simulink model "FOC"  (R2024b)
settings: Solver=FixedStepDiscrete  StartTime=0.0  StopTime=0.1  FixedStep=0.00005  RelTol=1e-3  EnableMultiTasking=on
InitFcn:
  | % Check we are building from the correct Build folder
  | expectedDir = 'FOC\Build';
  | currentDir  = pwd;
  | 
  | if ~contains(currentDir, expectedDir)
  |     error(['Wrong folder! You must run from the Build folder.' ...
  |            '\nCurrent: %s' ...
  |            '\nExpected path to contain: %s'], ...
  |            currentDir, expectedDir);
  | end
  | 
  | % Load all signals and parameters
  | loadall();
values from neighbouring files (symbols this model uses):
  RNTCBreakpoints = single([      534 546 559 572 585 599 613 628 643 658 674 690      707 724 742 760 779 798 818 838 860 881 904 927      951 975 1001 1027 1054 1081 1110 1139 1170 1201 1234 1267      1302 1337 1374 1412 1451 1492 1534 1577 1622 1668 1716 1765      1817 1869 1924 1981 2039 2100 2163 2227 2295 2364 2436 2511      2588 2668 2751 2837 2927 3019 3115 3215 3318 3425 3536 3651      3771 3895 4024 4158 42 ...(+565 chars)    [maps.m]
  TNTCTable = single([      125 124 123 122 121 120 119 118 117 116 115 114      113 112 111 110 109 108 107 106 105 104 103 102      101 100 99 98 97 96 95 94 93 92 91 90      89 88 87 86 85 84 83 82 81 80 79 78      77 76 75 74 73 72 71 70 69 68 67 66      65 64 63 62 61 60 59 58 57 56 55 54      53 52 51 50 49 48 47 46 45 44 43 42      41 40 39 38 37 36 35 34 33 32 31 30      29 28 27 26 25 24 23 22 21 20 19 ...(+227 chars)    [maps.m]
undefined symbols (not defined in the file or in its folder): BEnableLedBlink, BEnableMotor, BUseEstimatedPhaseW, fClockFrequency, fElectrical, ISoftwareOCPTrip, NADCCurrentGain, NADCOffsetPhaseU, NADCOffsetPhaseV, NADCOffsetPhaseW, VOpenLoopVoltage
libraries: simulink x8, stm32f4xxblockslib x5, stm32g4xxblockslib x2, stm32blockslib x1, myLib x1, simulink_extras x1
settings Model: STM32="{\"AnalogInput\":[{\"ID\":\"FOC:8\"},{\"ID\":\"FOC:615\"},{\"ID\":\"FOC:616\"}],\"TimerBlock\":{\"ID\":\"FOC:63\"},\"HardwareInterrupt\":{\"ID\":\"FOC:599\"},\"DigitalPortRead\":{\"ID\":\"FOC:54\"},\"DigitalPortWrite\":{\"ID\":\"FOC:6\"},\"PWMOutput\":{\"ID\":\"FOC:422\"}}"  Creator=sakee  LastModifiedBy=sakee
settings SolverCC: PositivePriorityOrder=on  AutoInsertRateTranBlk=on
settings OptimizationCC: EnhancedBackFolding=on  PassReuseOutputArgsAs=Individual arguments  ZeroExternalMemoryAtStartup=off  ZeroInternalMemoryAtStartup=off  MaxStackSize=512  OptimizeBlockOrder=speed  DifferentSizesBufferReuse=on  OptimizationCustomize=off  EfficientTunableParamExpr=on
settings DebuggingCC: MultiTaskDSMMsg=none  ParameterTunabilityLossMsg=error
settings HardwareCC: ProdBitPerPointer=32  ProdBitPerSizeT=32  ProdBitPerPtrDiffT=32  ProdLargestAtomicInteger=Long  ProdLargestAtomicFloat=Double  ProdWordSize=32  ProdLongLongMode=on  ProdHWDeviceType=ARM Compatible->ARM Cortex-M
settings SFSimCC: SimCustomInitializer=CurrentSense_EnableOPAMPs();  MATLABDynamicMemAlloc=off
settings SFSimCC: SimCustomHeaderCode=|
  | #include "task_profiler.h"
  | #include "current_sense_init.h"
settings SFSimCC: SimUserSources=|
  | task_profiler.c
  | current_sense_init.c
settings SFSimCC: SimUserIncludeDirs=|
  | Execution_time
  | Current_sensing
settings RTWCC: Description=Embedded Coder  SystemTargetFile=ert.tlc  HardwareBoard=STM32G4xx Based  TLCOptions="-aInlineSetEventsForThisBaseRateFcn=TLC_FALSE -aSuppressMultiTaskScheduler=TLC_FALSE   -aRateBasedStepFcn=1"  TemplateMakefile=ert_default_tmf  RTWUseSimCustomCode=on  CustomInitializer=CurrentSense_EnableOPAMPs();  Toolchain=GNU Tools for ARM Embedded Processors  BuildConfiguration=Debug
settings RTWCC: CustomHeaderCode=|
  | #include "task_profiler.h"
  | #include "current_sense_init.h"
settings RTWCC: CustomInclude=|
  | Execution_time
  | Current_sensing
settings RTWCC: CustomSource=|
  | task_profiler.c
  | current_sense_init.c
settings CodeAppCC: ForceParamTrailComments=on  IgnoreCustomStorageClasses=off  OperatorAnnotations=on  SimulinkDataObjDesc=on  SFDataObjDesc=on  InsertBlockDesc=on
settings ERTTargetCC: TargetLangStandard=C99 (ISO)  CodeReplacementLibrary=ARM Cortex-M  ExtModeTransport=3  ExtModeStaticAlloc=on  ExtModeStaticAllocSize=2048  ExtModeMexFile=ext_xcp  ExtModeIntrfLevel=Level2 - Open  InlinedParameterPlacement=Hierarchical

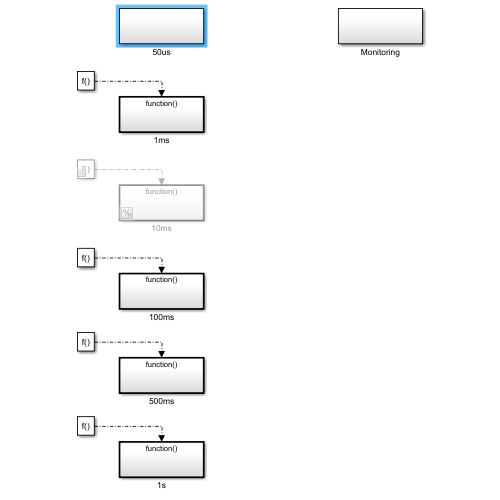
[thumbnail: Simulink's stored preview of the top-level diagram]
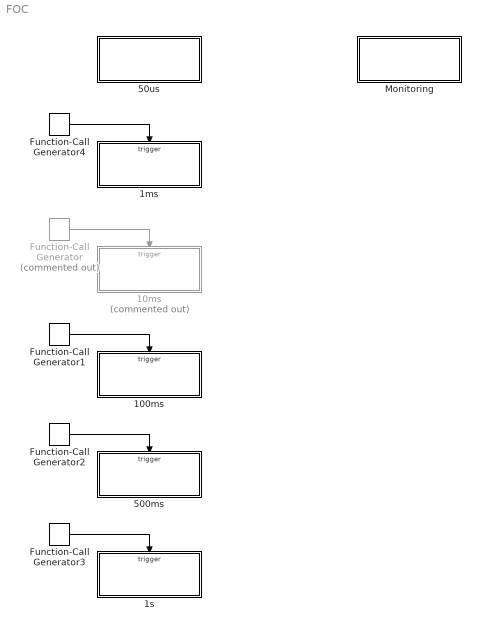
== system FOC ==
  100ms : Subsystem  TreatAsAtomicUnit=on
  10ms : Subsystem  Commented=on  TreatAsAtomicUnit=on
  1ms : Subsystem  TreatAsAtomicUnit=on
  1s : Subsystem  TreatAsAtomicUnit=on
  500ms : Subsystem  TreatAsAtomicUnit=on
  50us : Subsystem
  Function-Call Generator : simulink/Ports & Subsystems/Function-Call Generator  Commented=on  sample_time=0.01  numberOfIterations=1  DisallowWideOutput=off
  Function-Call Generator1 : simulink/Ports & Subsystems/Function-Call Generator  sample_time=0.1  numberOfIterations=1  DisallowWideOutput=off
  Function-Call Generator2 : simulink/Ports & Subsystems/Function-Call Generator  sample_time=0.5  numberOfIterations=1  DisallowWideOutput=off
  Function-Call Generator3 : simulink/Ports & Subsystems/Function-Call Generator  sample_time=1  numberOfIterations=1  DisallowWideOutput=off
  Function-Call Generator4 : simulink/Ports & Subsystems/Function-Call Generator  sample_time=0.001  numberOfIterations=1  DisallowWideOutput=off
  Monitoring : Subsystem
  wires:
  Function-Call Generator/1 -> 10ms/Trigger
  Function-Call Generator1/1 -> 100ms/Trigger
  Function-Call Generator3/1 -> 1s/Trigger
  Function-Call Generator2/1 -> 500ms/Trigger
  Function-Call Generator4/1 -> 1ms/Trigger

== system FOC/100ms ==
  function : TriggerPort  TriggerType=function-call  VariantControl=(inherit)
  COMP_States : Subsystem
  Init : Subsystem
  Sensors : Subsystem

== system FOC/10ms ==
  function : TriggerPort  TriggerType=function-call  VariantControl=(inherit)

== system FOC/1ms ==
  function : TriggerPort  TriggerType=function-call  VariantControl=(inherit)
  LED : Subsystem
  Motor Safety : Subsystem

== system FOC/1s ==
  function : TriggerPort  TriggerType=function-call  VariantControl=(inherit)
  Cast To Boolean : DataTypeConversion  OutDataTypeStr=boolean  SaturateOnIntegerOverflow=off  RndMeth=Floor
  Data Store Write1 : DataStoreWrite  DataStoreName=BLed1000ms  IndexOptions=Index vector (dialog)  Indices=1  OutputSizes=1
  Pulse Generator1 : DiscretePulseGenerator  SampleTime=-1
  wires:
  Pulse Generator1/1 -> Cast To Boolean/1
  Cast To Boolean/1 -> Data Store Write1/1

== system FOC/500ms ==
  function : TriggerPort  TriggerType=function-call  VariantControl=(inherit)
  Cast To Boolean : DataTypeConversion  OutDataTypeStr=boolean  SaturateOnIntegerOverflow=off  RndMeth=Floor
  Data Store Write1 : DataStoreWrite  DataStoreName=BLed500ms  IndexOptions=Index vector (dialog)  Indices=1  OutputSizes=1
  Pulse Generator1 : DiscretePulseGenerator  SampleTime=-1
  wires:
  Pulse Generator1/1 -> Cast To Boolean/1
  Cast To Boolean/1 -> Data Store Write1/1

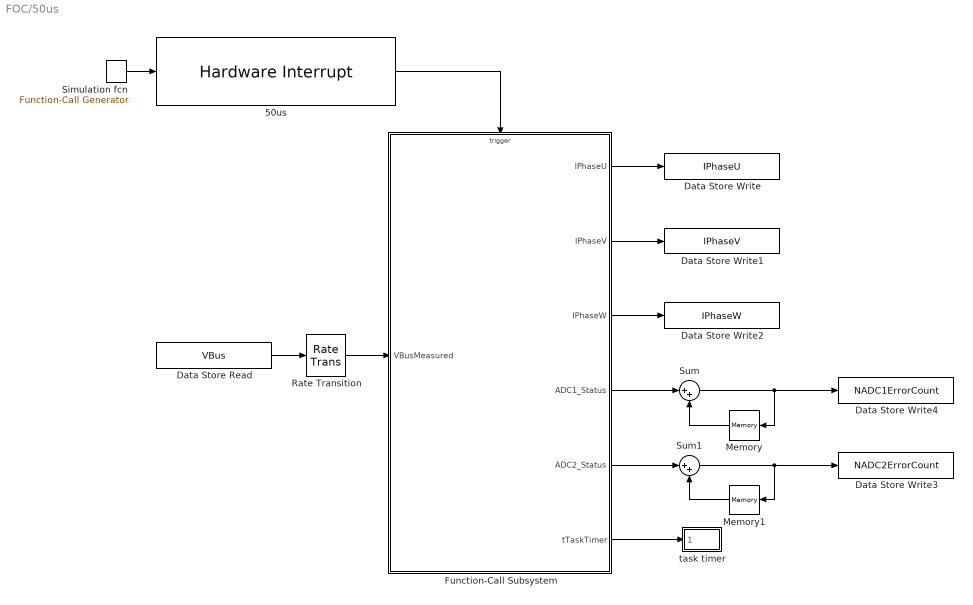
== system FOC/50us ==
  50us : stm32g4xxblockslib/Hardware Interrupt  ISRGroup=Analog to digital converter (ADC)  ISRName=ADC1_2_IRQHandler  ISRNumber=33  EventsList={ 'off', 'ADC1 OVR', '1'; 'off', 'ADC1 Reg EoCS', '2'; 'off', 'ADC1 Inj EoCS', '3'; 'off', 'ADC1 Inj JQOVF', '4'; 'off', 'ADC1 Watchdog1', '5'; 'off', 'ADC1 Watchdog2', '6'; 'off', 'ADC1 Watchdog3', '7'; 'off', 'ADC2 OVR', '8'; 'off', 'ADC2 Reg EoCS', '9'; 'on', 'ADC2 Inj EoCS', '10'; 'off', 'ADC2 Inj JQOVF', '11'; 'off', 'ADC2 Watchdog1', '12'; 'off', 'ADC2 Watchdog2', '13'; 'off', 'ADC2 Watchdog3', '14'; 'off', 'Custom event', '15' }  SelectedEvents={'ADC2 Inj EoCS'}  TaskPriority=30  DisablePreemption=off  ClearInterruptFlagsAtEndOfEvent=on  InterruptDefinitionFile=$(TARGET_ROOT)/registry/interrupts/STM32F4xxBased_interrupts.xml  HardwareBoard=STM32G4xx Based  EnableSimPort=on
  Data Store Read : DataStoreRead  DataStoreName=VBus  IndexOptions=Index vector (dialog)  Indices=1  OutputSizes=1
  Data Store Write : DataStoreWrite  DataStoreName=IPhaseU  IndexOptions=Index vector (dialog)  Indices=1  OutputSizes=1
  Data Store Write1 : DataStoreWrite  DataStoreName=IPhaseV  IndexOptions=Index vector (dialog)  Indices=1  OutputSizes=1
  Data Store Write2 : DataStoreWrite  DataStoreName=IPhaseW  IndexOptions=Index vector (dialog)  Indices=1  OutputSizes=1
  Data Store Write3 : DataStoreWrite  DataStoreName=NADC2ErrorCount  IndexOptions=Index vector (dialog)  Indices=1  OutputSizes=1
  Data Store Write4 : DataStoreWrite  DataStoreName=NADC1ErrorCount  IndexOptions=Index vector (dialog)  Indices=1  OutputSizes=1
  Function-Call Subsystem : Subsystem  TreatAsAtomicUnit=on
  Memory : Memory  InheritSampleTime=on
  Memory1 : Memory  InheritSampleTime=on
  Rate Transition : RateTransition  Deterministic=off
  Simulation fcn : simulink/Ports & Subsystems/Function-Call Generator  sample_time=50e-6  numberOfIterations=1  DisallowWideOutput=off
  Sum : Sum  Inputs=|++
  Sum1 : Sum  Inputs=|++
  task timer : Subsystem
  wires:
  Function-Call Subsystem/2(IPhaseV) -> Data Store Write1/1
  Function-Call Subsystem/4(ADC1_Status) -> Sum/1
  Function-Call Subsystem/1(IPhaseU) -> Data Store Write/1
  Function-Call Subsystem/3(IPhaseW) -> Data Store Write2/1
  Function-Call Subsystem/5(ADC2_Status) -> Sum1/1
  Sum1/1 -> Memory1/1, Data Store Write3/1
  Memory/1 -> Sum/2
  Sum/1 -> Data Store Write4/1, Memory/1
  Memory1/1 -> Sum1/2
  50us/1 -> Function-Call Subsystem/Trigger
  Simulation fcn/1 -> 50us/1
  Function-Call Subsystem/6(tTaskTimer) -> task timer/1(" ")
  Data Store Read/1 -> Rate Transition/1
  Rate Transition/1 -> Function-Call Subsystem/1(VBusMeasured)

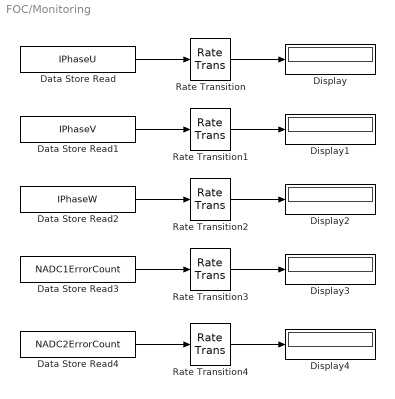
== system FOC/Monitoring ==
  Data Store Read : DataStoreRead  DataStoreName=IPhaseU  IndexOptions=Index vector (dialog)  Indices=1  OutputSizes=1
  Data Store Read1 : DataStoreRead  DataStoreName=IPhaseV  IndexOptions=Index vector (dialog)  Indices=1  OutputSizes=1
  Data Store Read2 : DataStoreRead  DataStoreName=IPhaseW  IndexOptions=Index vector (dialog)  Indices=1  OutputSizes=1
  Data Store Read3 : DataStoreRead  DataStoreName=NADC1ErrorCount  IndexOptions=Index vector (dialog)  Indices=1  OutputSizes=1
  Data Store Read4 : DataStoreRead  DataStoreName=NADC2ErrorCount  IndexOptions=Index vector (dialog)  Indices=1  OutputSizes=1
  Display{,1..4} (5 alike) : Display
  Rate Transition{,1..4} (5 alike) : RateTransition  OutPortSampleTime=0.1
  wires:
  Data Store Read/1 -> Rate Transition/1
  Data Store Read1/1 -> Rate Transition1/1
  Data Store Read2/1 -> Rate Transition2/1
  Rate Transition/1 -> Display/1
  Rate Transition1/1 -> Display1/1
  Rate Transition2/1 -> Display2/1
  Data Store Read3/1 -> Rate Transition3/1
  Data Store Read4/1 -> Rate Transition4/1
  Rate Transition3/1 -> Display3/1
  Rate Transition4/1 -> Display4/1

== system FOC/100ms/COMP_States ==
  C Caller : CCaller  FunctionName=CurrentSense_UpdateCOMPStates

== system FOC/100ms/Init ==
  note: Enable TIM2 timer, Used to trigger ADC1
  note: Blink LED
  Cast To Boolean : DataTypeConversion  OutDataTypeStr=boolean  SaturateOnIntegerOverflow=off  RndMeth=Floor
  Data Store Write1 : DataStoreWrite  DataStoreName=BLed100ms  IndexOptions=Index vector (dialog)  Indices=1  OutputSizes=1
  Pulse Generator1 : DiscretePulseGenerator  SampleTime=-1
  Terminator : Terminator
  Timer1 : stm32blockslib/Timer  TimerModule=TIM2  EnableFrequencyInput=off  EnableCounterInput=off  EnableMainOutputInput=off  SetRCAfterCE=off  OutputDirection=off  OutputMainOutputEnableStatus=off  SampleTime=-1  EnableUpdateEvent=off  EnableCaptureCompare1Event=off  EnableCaptureCompare2Event=off  EnableCaptureCompare3Event=off  EnableCaptureCompare4Event=off  EnableTriggerEvent=off  EnableBreakEvent=off  EnableBreakEvent2=off  EnableCOMGenerationEvent=off  ProcessorFamily=STM32G4
      settings: LibrarySourceBlock=stm32g4xxblockslib/Timer
  wires:
  Cast To Boolean/1 -> Data Store Write1/1
  Timer1/1 -> Terminator/1
  Pulse Generator1/1 -> Cast To Boolean/1

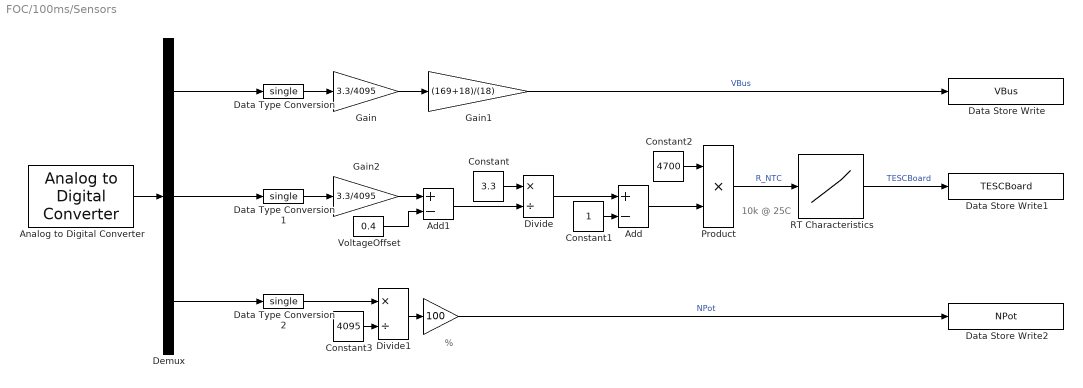
== system FOC/100ms/Sensors ==
  note: %
  note: 10k @ 25C
  " " : Gain  Gain=100  OutDataTypeStr=single
  Add : Sum  Inputs=+-
  Add1 : Sum  Inputs=+-
  Analog to Digital Converter : stm32f4xxblockslib/Analog to Digital Converter  ADCModule=ADC1  ConversionGroup=Regular  TriggerMode=Read results only  NumberOfConversions=3  EnableBufferConv=off  BufferLength=1  OutputStatus=off  SampleTime=-1  EnableSimPort=off  hoistedMaskSrc=ECSoC/ECSimCodegen/Analog to Digital Converter
  Constant : Constant  Value=3.3  OutDataTypeStr=single
  Constant1 : Constant  OutDataTypeStr=single
  Constant2 : Constant  Value=4700  OutDataTypeStr=single
  Constant3 : Constant  Value=4095  OutDataTypeStr=single
  Data Store Write : DataStoreWrite  DataStoreName=VBus  IndexOptions=Index vector (dialog)  Indices=1  OutputSizes=1
  Data Store Write1 : DataStoreWrite  DataStoreName=TESCBoard  IndexOptions=Index vector (dialog)  Indices=1  OutputSizes=1
  Data Store Write2 : DataStoreWrite  DataStoreName=NPot  IndexOptions=Index vector (dialog)  Indices=1  OutputSizes=1
  Data Type Conversion : DataTypeConversion  OutDataTypeStr=single  SaturateOnIntegerOverflow=off  RndMeth=Floor
  Data Type Conversion1 : DataTypeConversion  OutDataTypeStr=single  SaturateOnIntegerOverflow=off  RndMeth=Floor
  Data Type Conversion2 : DataTypeConversion  OutDataTypeStr=single  SaturateOnIntegerOverflow=off  RndMeth=Floor
  Demux : Demux  Outputs=3
  Divide : Product  Inputs=*/
  Divide1 : Product  Inputs=*/
  Gain : Gain  Gain=3.3/4095  OutDataTypeStr=single
  Gain1 : Gain  Gain=(169+18)/(18)  OutDataTypeStr=single
  Gain2 : Gain  Gain=3.3/4095  OutDataTypeStr=single
  Product : Product
  RT Characteristics : Lookup_n-D  NumberOfTableDimensions=1  BreakpointsForDimension1=RNTCBreakpoints  Table=TNTCTable  InternalRulePriority=Speed  RndMeth=Simplest
  VoltageOffset : Constant  Value=0.4  OutDataTypeStr=single
  wires:
  Gain/1 -> Gain1/1
  Analog to Digital Converter/1 -> Demux/1
  Demux/1 -> Data Type Conversion/1
  Data Type Conversion/1 -> Gain/1
  Demux/2 -> Data Type Conversion1/1
  Data Type Conversion1/1 -> Gain2/1
  Gain1/1 -> Data Store Write/1  "VBus"
  Constant/1 -> Divide/1
  Divide/1 -> Add/1
  Constant1/1 -> Add/2
  Product/1 -> RT Characteristics/1  "R_NTC"
  Constant2/1 -> Product/1
  Add/1 -> Product/2
  RT Characteristics/1 -> Data Store Write1/1  "TESCBoard"
  Gain2/1 -> Add1/1
  VoltageOffset/1 -> Add1/2
  Add1/1 -> Divide/2
  Data Type Conversion2/1 -> Divide1/1
  Demux/3 -> Data Type Conversion2/1
  Constant3/1 -> Divide1/2
  Divide1/1 -> " "/1
  " "/1 -> Data Store Write2/1  "NPot"

== system FOC/1ms/LED ==
  Compare To Constant : simulink/Logic and Bit Operations/Compare To Constant  relop=>  const=1  OutDataTypeStr=boolean
  Constant : Constant  Value=BEnableLedBlink
  Constant1 : Constant
  Data Store Read : DataStoreRead  DataStoreName=BLed100ms  IndexOptions=Index vector (dialog)  Indices=1  OutputSizes=1
  Data Store Read1 : DataStoreRead  DataStoreName=BLed500ms  IndexOptions=Index vector (dialog)  Indices=1  OutputSizes=1
  Data Store Read2 : DataStoreRead  DataStoreName=BLed1000ms  IndexOptions=Index vector (dialog)  Indices=1  OutputSizes=1
  Digital Port Read1 : stm32f4xxblockslib/Digital Port Read  PortName=GPIOC  PinNumber=[10]  ReadOperation=on  IOAsArray=on  SampleTime=-1  EnableSimPort=off  hoistedMaskSrc=ECSoC/ECSimCodegen/Digital Port Read
      settings: LibrarySourceBlock=stm32g4xxblockslib/Digital Port Read
  Digital Port Write : stm32f4xxblockslib/Digital Port Write  PortName=GPIOC  PinNumber=[6]  ReadOperation=off  IOAsArray=on  EnableSimPort=off  hoistedMaskSrc=ECSoC/ECSimCodegen/Digital Port Write
      settings: LibrarySourceBlock=stm32g4xxblockslib/Digital Port Write
  Function-Call Subsystem : Subsystem  TreatAsAtomicUnit=on
  Ground : Ground
  Logical Operator : Logic  AllPortsSameDT=off  OutDataTypeStr=boolean
  Multiport Switch : MultiPortSwitch  DataPortOrder=Zero-based contiguous  zeroidx=on  SaturateOnIntegerOverflow=off  InputSameDT=off
  Switch : Switch  Criteria=u2 > Threshold  SaturateOnIntegerOverflow=off  InputSameDT=off
  Timer : myLib/Timer  tSampleTime=0.001
  wires:
  Data Store Read2/1 -> Multiport Switch/4
  Function-Call Subsystem/1(Out1) -> Multiport Switch/1
  Compare To Constant/1 -> Switch/3, Switch/2
  Data Store Read1/1 -> Multiport Switch/3
  Constant1/1 -> Timer/1
  Switch/1 -> Logical Operator/2
  Constant/1 -> Switch/1
  Digital Port Read1/1 -> Function-Call Subsystem/Trigger
  Multiport Switch/1 -> Logical Operator/1
  Logical Operator/1 -> Digital Port Write/1
  Ground/1 -> Timer/2
  Timer/1 -> Compare To Constant/1
  Data Store Read/1 -> Multiport Switch/2

== system FOC/1ms/Motor Safety ==
  C Caller2 : CCaller  FunctionName=MotorSafety_SetMOE  PortSpecificationStruct="%)30     .    R ,   8    (     @         %    \"     (    !     0         %  0 \"0    $    _    07)G3F%M90  4&]R=$YA;64 4V-O<&4     26YD97@     5'EP90      4VEZ90      27-';&]B86P   X    P    !@    @    $          4    (     0    ,    !         !   P!O=70 #@   #     &    \"     0         !0    @    !     P    $         $  # &]U=  .    .     8    (    !          %    \"     $    &     0         0    !@   $]U='!U=   #@   #@    &    \"     8         !0    @    !     0    $         \"0    @               X    X    !@    @    $          4    (     0    4    !         !     %    =6EN=#@    .    ,     8    (    !          %    \"     $    !     0         0  $ ,0    X    P    !@    @    ) @        4    (     0    $    !          (  0      #@   #@    &    \"     0         !0    @    !    !@    $         $     8   !E;F%B;&4   X    X    !@    @    $          4    (     0    8    !         !     &    96YA8FQE   .    .     8    (    !          %    \"     $    %     0         0    !0   $EN<'5T    #@   #@    &    \"     8         !0    @    !     0    $         \"0    @               X    X    !@    @    $          4    (     0    4    !         !     %    =6EN=#@    .    ,     8    (    !          %    \"     $    !     0         0  $ ,0    X    P    !@    @    ) @        4    (     0    $    !          (  0"
  Data Store Write5 : DataStoreWrite  DataStoreName=BMotorOutputEnabled  IndexOptions=Index vector (dialog)  Indices=1  OutputSizes=1
  Data Type Conversion1 : DataTypeConversion  OutDataTypeStr=uint8  SaturateOnIntegerOverflow=off  RndMeth=Floor
  Data Type Conversion2 : DataTypeConversion  OutDataTypeStr=uint8  SaturateOnIntegerOverflow=off  RndMeth=Floor
  Subsystem : Subsystem
  wires:
  Data Type Conversion1/1 -> Data Store Write5/1
  C Caller2/1 -> Data Type Conversion1/1
  Subsystem/1(BMotorArmed) -> Data Type Conversion2/1
  Data Type Conversion2/1 -> C Caller2/1

== system FOC/50us/Function-Call Subsystem ==
  VBusMeasured : Inport
  function : TriggerPort  TriggerType=function-call  VariantControl=(inherit)
  C Caller : CCaller  ExecutionOrder=First  FunctionName=Profiler_FOC_Start
  C Caller1 : CCaller  ExecutionOrder=Last  FunctionName=Profiler_FOC_Stop  PortSpecificationStruct="%)30     .    & (   8    (     @         %    \"     $    !     0         %  0 \"0    $    _    07)G3F%M90  4&]R=$YA;64 4V-O<&4     26YD97@     5'EP90      4VEZ90      27-';&]B86P   X    P    !@    @    $          4    (     0    ,    !         !   P!O=70 #@   #     &    \"     0         !0    @    !     P    $         $  # &]U=  .    .     8    (    !          %    \"     $    &     0         0    !@   $]U='!U=   #@   #@    &    \"     8         !0    @    !     0    $         \"0    @               X    X    !@    @    $          4    (     0    8    !         !     &    =6EN=#,R   .    ,     8    (    !          %    \"     $    !     0         0  $ ,0    X    P    !@    @    ) @        4    (     0    $    !          (  0"
  FOC : Subsystem  TreatAsAtomicUnit=on
  Phase Current : Subsystem
  IPhaseU : Outport
  IPhaseV : Outport  Port=2
  IPhaseW : Outport  Port=3
  ADC1_Status : Outport  Port=4
  ADC2_Status : Outport  Port=5
  tTaskTimer : Outport  Port=6
  wires:
  Phase Current/1(IPhaseU) -> FOC/1(IPhaseU), IPhaseU/1
  Phase Current/2(IPhaseV) -> FOC/2(IPhaseV), IPhaseV/1
  Phase Current/3(IPhaseW) -> FOC/3(IPhaseW), IPhaseW/1
  Phase Current/4(ADC1_Status) -> ADC1_Status/1
  Phase Current/5(ADC2_Status) -> ADC2_Status/1
  C Caller1/1 -> tTaskTimer/1
  VBusMeasured/1 -> FOC/4(VBusMeasured)

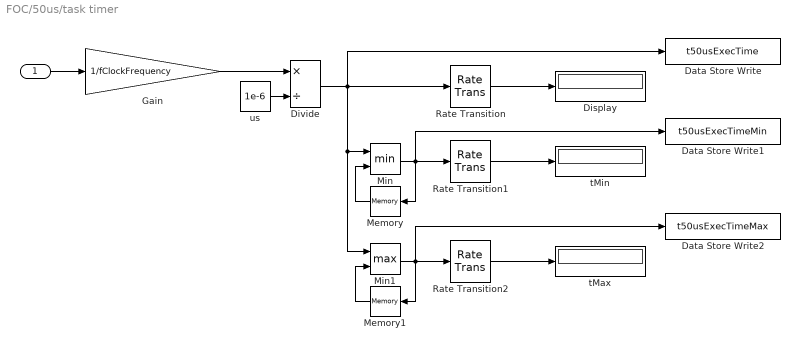
== system FOC/50us/task timer ==
  " " : Inport
  Data Store Write : DataStoreWrite  DataStoreName=t50usExecTime  IndexOptions=Index vector (dialog)  Indices=1  OutputSizes=1
  Data Store Write1 : DataStoreWrite  DataStoreName=t50usExecTimeMin  IndexOptions=Index vector (dialog)  Indices=1  OutputSizes=1
  Data Store Write2 : DataStoreWrite  DataStoreName=t50usExecTimeMax  IndexOptions=Index vector (dialog)  Indices=1  OutputSizes=1
  Display : Display
  Divide : Product  Inputs=*/
  Gain : Gain  Gain=1/fClockFrequency
  Memory : Memory  InitialCondition=inf  InheritSampleTime=on
  Memory1 : Memory  InheritSampleTime=on
  Min : MinMax  Inputs=2
  Min1 : MinMax  Function=max  Inputs=2
  Rate Transition : RateTransition  OutPortSampleTime=1
  Rate Transition1 : RateTransition  OutPortSampleTime=1
  Rate Transition2 : RateTransition  OutPortSampleTime=1
  tMax : Display
  tMin : Display
  us : Constant  Value=1e-6  OutDataTypeStr=single
  wires:
  " "/1 -> Gain/1
  Gain/1 -> Divide/1
  us/1 -> Divide/2
  Min/1 -> Data Store Write1/1, Memory/1, Rate Transition1/1
  Memory/1 -> Min/2
  Min1/1 -> Data Store Write2/1, Rate Transition2/1, Memory1/1
  Memory1/1 -> Min1/2
  Rate Transition/1 -> Display/1
  Divide/1 -> Data Store Write/1, Rate Transition/1, Min1/1, Min/1
  Rate Transition1/1 -> tMin/1
  Rate Transition2/1 -> tMax/1

== system FOC/1ms/LED/Function-Call Subsystem ==
  Trigger : TriggerPort  VariantControl=(inherit)  PortDimensions=1
  Repeating Sequence Stair : simulink/Sources/Repeating Sequence Stair  OutValues=[1 2 0]  tsamp=-1  OutMin=[]  OutMax=[]  OutDataTypeStr=double  OutputDataTypeScalingMode=double  OutDataType=fixdt(0,8)  ConRadixGroup=Best Precision: Vector-wise  OutScaling=2^-12
  Out1 : Outport
  wires:
  Repeating Sequence Stair/1 -> Out1/1

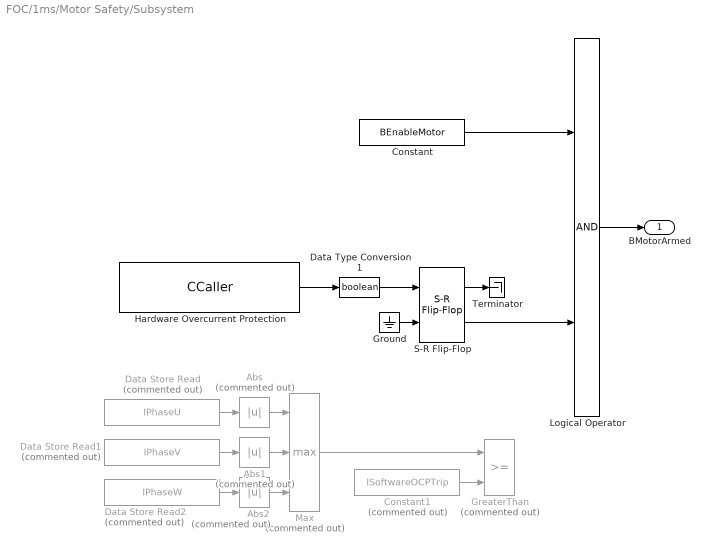
== system FOC/1ms/Motor Safety/Subsystem ==
  Abs : Abs  Commented=on  SaturateOnIntegerOverflow=off
  Abs1 : Abs  Commented=on  SaturateOnIntegerOverflow=off
  Abs2 : Abs  Commented=on  SaturateOnIntegerOverflow=off
  Constant : Constant  Value=BEnableMotor  OutDataTypeStr=boolean
  Constant1 : Constant  Commented=on  Value=ISoftwareOCPTrip  OutDataTypeStr=boolean
  Data Store Read : DataStoreRead  Commented=on  DataStoreName=IPhaseU  IndexOptions=Index vector (dialog)  Indices=1  OutputSizes=1
  Data Store Read1 : DataStoreRead  Commented=on  DataStoreName=IPhaseV  IndexOptions=Index vector (dialog)  Indices=1  OutputSizes=1
  Data Store Read2 : DataStoreRead  Commented=on  DataStoreName=IPhaseW  IndexOptions=Index vector (dialog)  Indices=1  OutputSizes=1
  Data Type Conversion1 : DataTypeConversion  OutDataTypeStr=boolean  SaturateOnIntegerOverflow=off  RndMeth=Floor
  GreaterThan : RelationalOperator  Commented=on  OutDataTypeStr=boolean  RndMeth=Simplest  InputSameDT=off
  Ground : Ground
  Hardware Overcurrent Protection : CCaller  FunctionName=MotorSafety_GetHardwareFault  PortSpecificationStruct="%)30     .    & (   8    (     @         %    \"     $    !     0         %  0 \"0    $    _    07)G3F%M90  4&]R=$YA;64 4V-O<&4     26YD97@     5'EP90      4VEZ90      27-';&]B86P   X    P    !@    @    $          4    (     0    ,    !         !   P!O=70 #@   #     &    \"     0         !0    @    !     P    $         $  # &]U=  .    .     8    (    !          %    \"     $    &     0         0    !@   $]U='!U=   #@   #@    &    \"     8         !0    @    !     0    $         \"0    @               X    X    !@    @    $          4    (     0    4    !         !     %    =6EN=#@    .    ,     8    (    !          %    \"     $    !     0         0  $ ,0    X    P    !@    @    ) @        4    (     0    $    !          (  0"
  Logical Operator : Logic  AllPortsSameDT=off  OutDataTypeStr=boolean
  Max : MinMax  Commented=on  Function=max  Inputs=3
  S-R Flip-Flop : simulink_extras/Flip Flops/S-R Flip-Flop  initial_condition=0
  Terminator : Terminator
  BMotorArmed : Outport
  wires:
  Logical Operator/1 -> BMotorArmed/1
  Ground/1 -> S-R Flip-Flop/2
  S-R Flip-Flop/1 -> Terminator/1
  Data Type Conversion1/1 -> S-R Flip-Flop/1
  Constant/1 -> Logical Operator/1
  Data Store Read/1 -> Abs/1
  Data Store Read1/1 -> Abs1/1
  Data Store Read2/1 -> Abs2/1
  Hardware Overcurrent Protection/1 -> Data Type Conversion1/1
  Max/1 -> GreaterThan/1
  Abs/1 -> Max/1
  Abs1/1 -> Max/2
  Abs2/1 -> Max/3
  Constant1/1 -> GreaterThan/2
  S-R Flip-Flop/2 -> Logical Operator/2

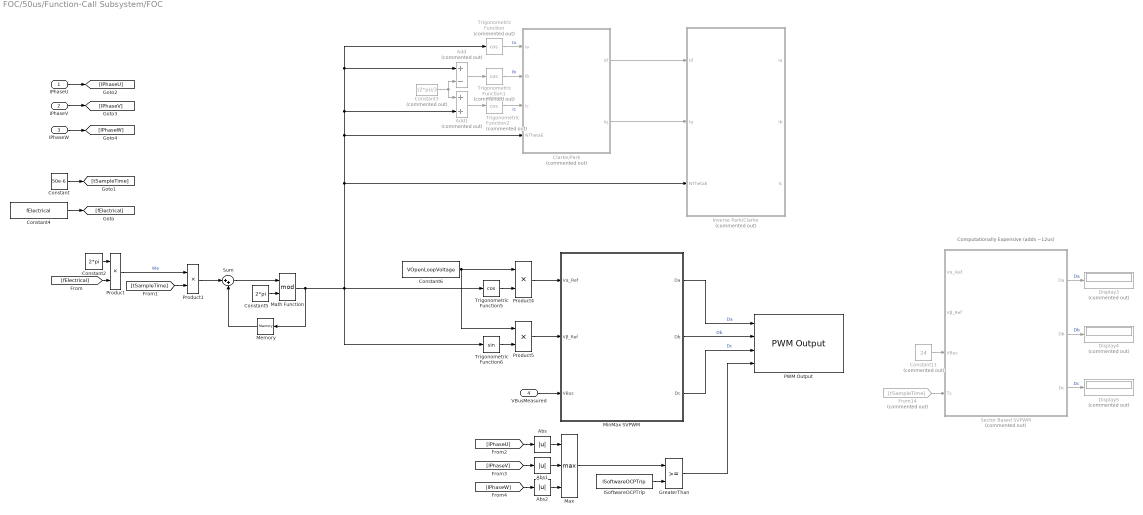
== system FOC/50us/Function-Call Subsystem/FOC ==
  note: Computationally Expensive (adds ~12us)
  IPhaseU : Inport
  IPhaseV : Inport  Port=2
  IPhaseW : Inport  Port=3
  VBusMeasured : Inport  Port=4
  Abs : Abs  SaturateOnIntegerOverflow=off
  Abs1 : Abs  SaturateOnIntegerOverflow=off
  Abs2 : Abs  SaturateOnIntegerOverflow=off
  Add : Sum  Commented=on  Inputs=+-
  Add1 : Sum  Commented=on
  Clarke/Park : Subsystem  Commented=on
  Constant : Constant  Value=50e-6  OutDataTypeStr=single
  Constant11 : Constant  Commented=on  Value=24  OutDataTypeStr=single
  Constant2 : Constant  Value=2*pi  OutDataTypeStr=single
  Constant3 : Constant  Commented=on  Value=(2*pi)/3  OutDataTypeStr=single
  Constant4 : Constant  Value=fElectrical  OutDataTypeStr=single
  Constant5 : Constant  Value=2*pi  OutDataTypeStr=single
  Constant6 : Constant  Value=VOpenLoopVoltage  OutDataTypeStr=single
  Display3 : Display  Commented=on
  Display4 : Display  Commented=on
  Display5 : Display  Commented=on
  From14 : From  Commented=on  GotoTag=tSampleTime
  GreaterThan : RelationalOperator  OutDataTypeStr=boolean  RndMeth=Simplest  InputSameDT=off
  ISoftwareOCPTrip : Constant  Value=ISoftwareOCPTrip  OutDataTypeStr=boolean
  Inverse Park/Clarke : Subsystem  Commented=on
  Math Function : Math  Operator=mod
  Max : MinMax  Function=max  Inputs=3
  Memory : Memory  InheritSampleTime=on
  MinMax SVPWM : Subsystem
  PWM Output : stm32g4xxblockslib/PWM Output  TimerModule=TIM1  DutycycleUnits=Percentage  EnableChannel1=on  EnableChannel2=on  EnableChannel3=on  EnableChannel4=off  EnableChannel5=off  EnableChannel6=off  EnableCounterInput=off  EnableMainOutputInput=off  EnableFrequencyInput=off  SetRCAfterCE=off  OutputDirection=off  OutputMainOutputEnableStatus=off  SampleTime=0.1  EnableSimPort=off  EnableUpdateEvent=off  EnableCaptureCompare1Event=off  EnableCaptureCompare2Event=off  EnableCaptureCompare3Event=off  EnableCaptureCompare4Event=off  EnableTriggerEvent=off  EnableBreakEvent=on  EnableBreakEvent2=off  ProcessorFamily=STM32G4  hoistedMaskSrc=ECSoC/ECSimCodegen/PWM Output
  Product{,1,4..5} (4 alike) : Product
  Sector Based SVPWM : Subsystem  Commented=on
  Sum : Sum  Inputs=|++
  Trigonometric Function : Trigonometry  Commented=on  Operator=cos
  Trigonometric Function1 : Trigonometry  Commented=on  Operator=cos
  Trigonometric Function2 : Trigonometry  Commented=on  Operator=cos
  Trigonometric Function5 : Trigonometry  Operator=cos
  Trigonometric Function6 : Trigonometry
  wires:
  Constant/1 -> [tSampleTime]
  Constant2/1 -> Product/1
  [fElectrical] -> Product/2
  Product/1 -> Product1/1  "We"
  [tSampleTime] -> Product1/2
  Product1/1 -> Sum/1
  Trigonometric Function/1 -> Clarke/Park/1(Ia)  "Ia"
  Add/1 -> Trigonometric Function1/1
  Constant3/1 -> Add/2, Add1/1
  Add1/1 -> Trigonometric Function2/1
  Trigonometric Function1/1 -> Clarke/Park/2(Ib)  "Ib"
  Trigonometric Function2/1 -> Clarke/Park/3(Ic)  "Ic"
  Constant11/1 -> Sector Based SVPWM/3(VBus)
  From14/1 -> Sector Based SVPWM/4(Ts)
  Constant5/1 -> Math Function/2
  Sum/1 -> Math Function/1
  Memory/1 -> Sum/2
  Abs1/1 -> Max/2
  ISoftwareOCPTrip/1 -> GreaterThan/2
  [IPhaseV] -> Abs1/1
  Max/1 -> GreaterThan/1
  [IPhaseW] -> Abs2/1
  [IPhaseU] -> Abs/1
  Abs2/1 -> Max/3
  Abs/1 -> Max/1
  IPhaseU/1 -> [IPhaseU]
  IPhaseV/1 -> [IPhaseV]
  IPhaseW/1 -> [IPhaseW]
  Sector Based SVPWM/1(Da) -> Display3/1  "Da"
  Sector Based SVPWM/2(Db) -> Display4/1  "Db"
  Sector Based SVPWM/3(Dc) -> Display5/1  "Dc"
  Trigonometric Function6/1 -> Product5/2
  Constant6/1 -> Product4/1, Product5/1
  Trigonometric Function5/1 -> Product4/2
  Math Function/1 -> Trigonometric Function6/1, Trigonometric Function5/1, Clarke/Park/4(NThetaE), Trigonometric Function/1, Add/1, Add1/2, Inverse Park/Clarke/3(NThetaE), Memory/1
  Clarke/Park/1(Id) -> Inverse Park/Clarke/1(Id)
  Clarke/Park/2(Iq) -> Inverse Park/Clarke/2(Iq)
  GreaterThan/1 -> PWM Output/4
  Product4/1 -> MinMax SVPWM/1(Vα_Ref)
  Product5/1 -> MinMax SVPWM/2(Vβ_Ref)
  MinMax SVPWM/1(Da) -> PWM Output/1  "Da"
  MinMax SVPWM/2(Db) -> PWM Output/2  "Db"
  MinMax SVPWM/3(Dc) -> PWM Output/3  "Dc"
  VBusMeasured/1 -> MinMax SVPWM/3(VBus)
  Constant4/1 -> [fElectrical]

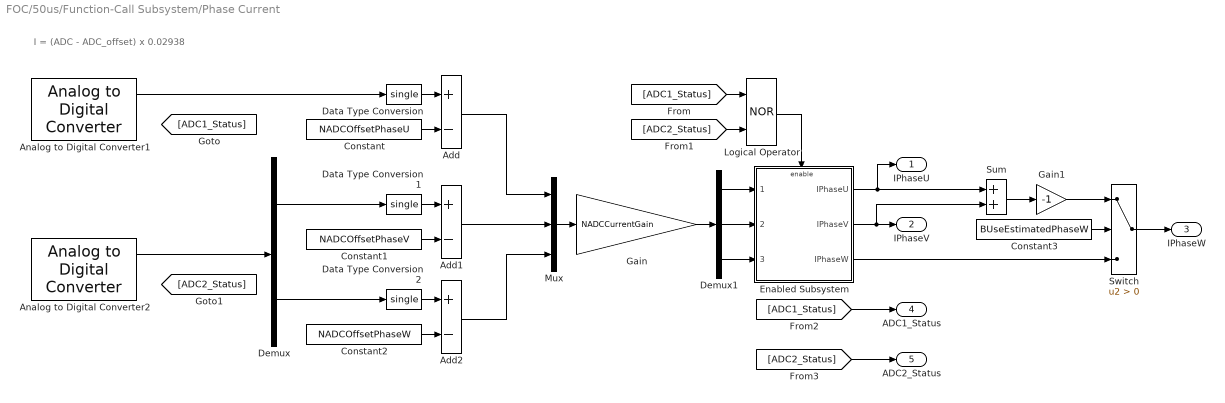
== system FOC/50us/Function-Call Subsystem/Phase Current ==
  note: I = (ADC - ADC_offset) x 0.02938
  Add : Sum  Inputs=+-
  Add1 : Sum  Inputs=+-
  Add2 : Sum  Inputs=+-
  Analog to Digital Converter1 : stm32f4xxblockslib/Analog to Digital Converter  ADCModule=ADC1  ConversionGroup=Injected  TriggerMode=Read results only  NumberOfConversions=1  EnableBufferConv=off  BufferLength=1  OutputStatus=on  SampleTime=-1  EnableSimPort=off  hoistedMaskSrc=ECSoC/ECSimCodegen/Analog to Digital Converter
  Analog to Digital Converter2 : stm32f4xxblockslib/Analog to Digital Converter  ADCModule=ADC2  ConversionGroup=Injected  TriggerMode=Read results only  NumberOfConversions=2  EnableBufferConv=off  BufferLength=1  OutputStatus=on  SampleTime=-1  EnableSimPort=off  hoistedMaskSrc=ECSoC/ECSimCodegen/Analog to Digital Converter
  Constant : Constant  Value=NADCOffsetPhaseU  OutDataTypeStr=single
  Constant1 : Constant  Value=NADCOffsetPhaseV  OutDataTypeStr=single
  Constant2 : Constant  Value=NADCOffsetPhaseW  OutDataTypeStr=single
  Constant3 : Constant  Value=BUseEstimatedPhaseW  OutDataTypeStr=boolean
  Data Type Conversion : DataTypeConversion  OutDataTypeStr=single  SaturateOnIntegerOverflow=off  RndMeth=Floor
  Data Type Conversion1 : DataTypeConversion  OutDataTypeStr=single  SaturateOnIntegerOverflow=off  RndMeth=Floor
  Data Type Conversion2 : DataTypeConversion  OutDataTypeStr=single  SaturateOnIntegerOverflow=off  RndMeth=Floor
  Demux : Demux  Outputs=2
  Demux1 : Demux  Outputs=3
  Enabled Subsystem : Subsystem  TreatAsAtomicUnit=on
  Gain : Gain  Gain=NADCCurrentGain
  Gain1 : Gain  Gain=-1
  Logical Operator : Logic  Operator=NOR  AllPortsSameDT=off  OutDataTypeStr=boolean
  Mux : Mux  Inputs=3
  Sum : Sum
  Switch : Switch  Criteria=u2 > Threshold  SaturateOnIntegerOverflow=off  InputSameDT=off
  IPhaseU : Outport
  IPhaseV : Outport  Port=2
  IPhaseW : Outport  Port=3
  ADC1_Status : Outport  Port=4
  ADC2_Status : Outport  Port=5
  wires:
  Analog to Digital Converter1/1 -> Data Type Conversion/1
  Demux/1 -> Data Type Conversion1/1
  Analog to Digital Converter2/1 -> Demux/1
  Demux/2 -> Data Type Conversion2/1
  Data Type Conversion/1 -> Add/1
  Constant/1 -> Add/2
  Constant1/1 -> Add1/2
  Data Type Conversion1/1 -> Add1/1
  Constant2/1 -> Add2/2
  Data Type Conversion2/1 -> Add2/1
  Add/1 -> Mux/1
  Add1/1 -> Mux/2
  Add2/1 -> Mux/3
  Mux/1 -> Gain/1
  Gain/1 -> Demux1/1
  ? -> [ADC1_Status]
  ? -> [ADC2_Status]
  [ADC1_Status] -> Logical Operator/1
  [ADC2_Status] -> Logical Operator/2
  Demux1/1 -> Enabled Subsystem/1(" ")
  Demux1/2 -> Enabled Subsystem/2("  ")
  Demux1/3 -> Enabled Subsystem/3("   ")
  [ADC1_Status] -> ADC1_Status/1
  [ADC2_Status] -> ADC2_Status/1
  Logical Operator/1 -> Enabled Subsystem/Enable
  Enabled Subsystem/1(IPhaseU) -> IPhaseU/1, Sum/1
  Enabled Subsystem/2(IPhaseV) -> Sum/2, IPhaseV/1
  Switch/1 -> IPhaseW/1
  Constant3/1 -> Switch/2
  Enabled Subsystem/3(IPhaseW) -> Switch/3
  Gain1/1 -> Switch/1
  Sum/1 -> Gain1/1

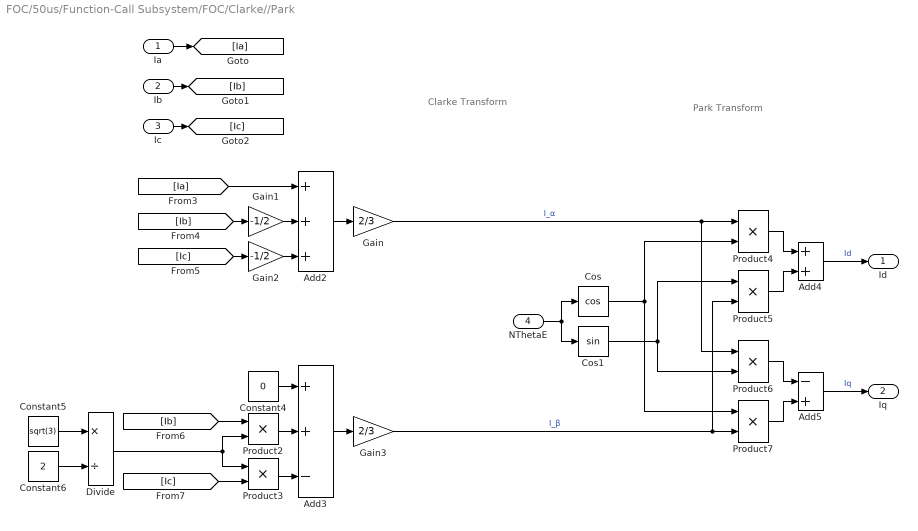
== system FOC/50us/Function-Call Subsystem/FOC/Clarke//Park ==
  note: Clarke Transform
  note: Park Transform
  Ia : Inport
  Ib : Inport  Port=2
  Ic : Inport  Port=3
  NThetaE : Inport  Port=4
  Add2 : Sum  Inputs=+++
  Add3 : Sum  Inputs=++-
  Add4 : Sum
  Add5 : Sum  Inputs=-+
  Constant4 : Constant  Value=0  OutDataTypeStr=single
  Constant5 : Constant  Value=sqrt(3)  OutDataTypeStr=single
  Constant6 : Constant  Value=2  OutDataTypeStr=single
  Cos : Trigonometry  Operator=cos
  Cos1 : Trigonometry
  Divide : Product  Inputs=*/
  Gain : Gain  Gain=2/3
  Gain1 : Gain  Gain=-1/2
  Gain2 : Gain  Gain=-1/2
  Gain3 : Gain  Gain=2/3
  Product{2..7} (6 alike) : Product
  Id : Outport
  Iq : Outport  Port=2
  wires:
  Product3/1 -> Add3/3
  [Ic] -> Gain2/1
  Add2/1 -> Gain/1
  [Ia] -> Add2/1
  Add4/1 -> Id/1  "Id"
  Constant5/1 -> Divide/1
  Add5/1 -> Iq/1  "Iq"
  [Ib] -> Gain1/1
  Constant4/1 -> Add3/1
  Add3/1 -> Gain3/1
  Cos1/1 -> Product5/1, Product6/2
  Product6/1 -> Add5/1
  Gain2/1 -> Add2/3
  Cos/1 -> Product4/2, Product7/1
  Product2/1 -> Add3/2
  Gain1/1 -> Add2/2
  Product4/1 -> Add4/1
  Constant6/1 -> Divide/2
  Product7/1 -> Add5/2
  Product5/1 -> Add4/2
  Gain/1 -> Product4/1, Product6/1  "I_α"
  Divide/1 -> Product2/2, Product3/1
  [Ib] -> Product2/1
  NThetaE/1 -> Cos/1, Cos1/1
  Gain3/1 -> Product7/2, Product5/2  "I_β"
  [Ic] -> Product3/2
  Ia/1 -> [Ia]
  Ib/1 -> [Ib]
  Ic/1 -> [Ic]

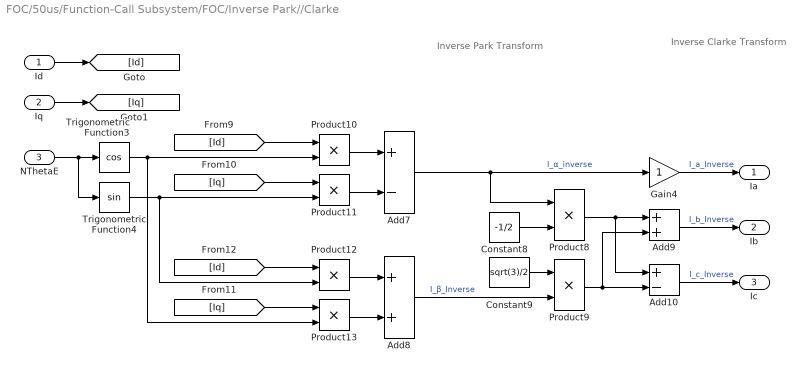
== system FOC/50us/Function-Call Subsystem/FOC/Inverse Park//Clarke ==
  note: Inverse Park Transform
  note: Inverse Clarke Transform
  Id : Inport
  Iq : Inport  Port=2
  NThetaE : Inport  Port=3
  Add10 : Sum  Inputs=+-
  Add7 : Sum  Inputs=+-
  Add8 : Sum
  Add9 : Sum
  Constant8 : Constant  Value=-1/2  OutDataTypeStr=single
  Constant9 : Constant  Value=sqrt(3)/2  OutDataTypeStr=single
  Gain4 : Gain
  Product{8..13} (6 alike) : Product
  Trigonometric Function3 : Trigonometry  Operator=cos
  Trigonometric Function4 : Trigonometry
  Ia : Outport
  Ib : Outport  Port=2
  Ic : Outport  Port=3
  wires:
  [Id] -> Product12/1
  Product12/1 -> Add8/1
  Trigonometric Function4/1 -> Product12/2, Product11/2
  Add8/1 -> Product9/2  "I_β_Inverse"
  [Iq] -> Product11/1
  Product11/1 -> Add7/2
  Constant8/1 -> Product8/2
  Product10/1 -> Add7/1
  Add9/1 -> Ib/1  "I_b_Inverse"
  Product13/1 -> Add8/2
  Product9/1 -> Add10/2, Add9/2
  Product8/1 -> Add9/1, Add10/1
  Add7/1 -> Gain4/1, Product8/1  "I_α_inverse"
  Constant9/1 -> Product9/1
  [Iq] -> Product13/1
  Gain4/1 -> Ia/1  "I_a_Inverse"
  [Id] -> Product10/1
  Add10/1 -> Ic/1  "I_c_Inverse"
  NThetaE/1 -> Trigonometric Function3/1, Trigonometric Function4/1
  Trigonometric Function3/1 -> Product13/2, Product10/2
  Id/1 -> [Id]
  Iq/1 -> [Iq]

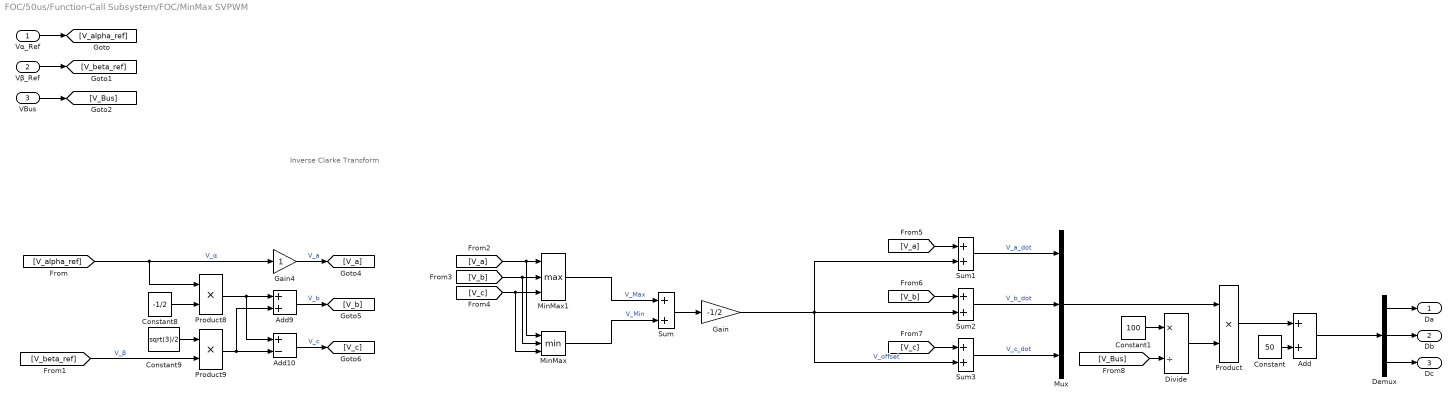
== system FOC/50us/Function-Call Subsystem/FOC/MinMax SVPWM ==
  note: Inverse Clarke Transform
  Vα_Ref : Inport
  Vβ_Ref : Inport  Port=2
  VBus : Inport  Port=3
  Add : Sum
  Add10 : Sum  Inputs=+-
  Add9 : Sum
  Constant : Constant  Value=50  OutDataTypeStr=single
  Constant1 : Constant  Value=100  OutDataTypeStr=single
  Constant8 : Constant  Value=-1/2  OutDataTypeStr=single
  Constant9 : Constant  Value=sqrt(3)/2  OutDataTypeStr=single
  Demux : Demux  Outputs=3
  Divide : Product  Inputs=*/
  Gain : Gain  Gain=-1/2
  Gain4 : Gain
  MinMax : MinMax  Inputs=3
  MinMax1 : MinMax  Function=max  Inputs=3
  Mux : Mux  Inputs=3
  Product : Product
  Product8 : Product
  Product9 : Product
  Sum{,1..3} (4 alike) : Sum
  Da : Outport
  Db : Outport  Port=2
  Dc : Outport  Port=3
  wires:
  VBus/1 -> [V_Bus]
  Vβ_Ref/1 -> [V_beta_ref]
  Vα_Ref/1 -> [V_alpha_ref]
  [V_beta_ref] -> Product9/2  "V_β"
  Constant8/1 -> Product8/2
  Constant9/1 -> Product9/1
  Product8/1 -> Add9/1, Add10/1
  Product9/1 -> Add10/2, Add9/2
  [V_alpha_ref] -> Gain4/1, Product8/1  "V_α"
  MinMax1/1 -> Sum/1  "V_Max"
  MinMax/1 -> Sum/2  "V_Min"
  Sum/1 -> Gain/1
  Gain4/1 -> [V_a]  "V_a"
  Add9/1 -> [V_b]  "V_b"
  Add10/1 -> [V_c]  "V_c"
  [V_a] -> MinMax/1, MinMax1/1
  [V_b] -> MinMax/2, MinMax1/2
  [V_c] -> MinMax/3, MinMax1/3
  [V_a] -> Sum1/1
  Gain/1 -> Sum3/2, Sum2/2, Sum1/2  "V_offset"
  [V_b] -> Sum2/1
  [V_c] -> Sum3/1
  Constant/1 -> Add/2
  Divide/1 -> Product/2
  [V_Bus] -> Divide/2
  Constant1/1 -> Divide/1
  Product/1 -> Add/1
  Mux/1 -> Product/1
  Demux/1 -> Da/1
  Demux/2 -> Db/1
  Demux/3 -> Dc/1
  Add/1 -> Demux/1
  Sum2/1 -> Mux/2  "V_b_dot"
  Sum1/1 -> Mux/1  "V_a_dot"
  Sum3/1 -> Mux/3  "V_c_dot"

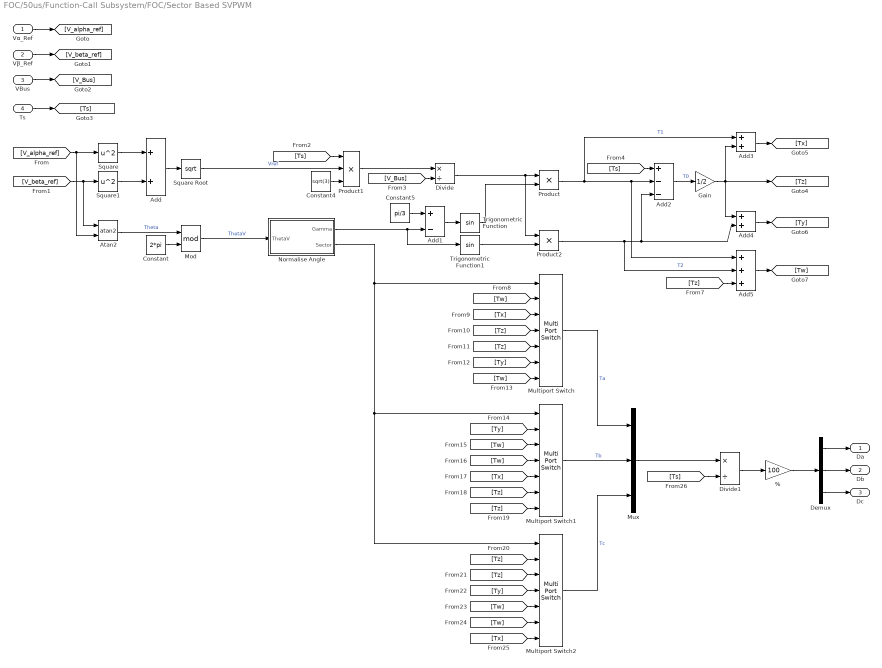
== system FOC/50us/Function-Call Subsystem/FOC/Sector Based SVPWM ==
  Vα_Ref : Inport
  Vβ_Ref : Inport  Port=2
  VBus : Inport  Port=3
  Ts : Inport  Port=4
  % : Gain  Gain=100
  Add : Sum
  Add1 : Sum  Inputs=+-
  Add2 : Sum  Inputs=+--
  Add3 : Sum
  Add4 : Sum
  Add5 : Sum  Inputs=+++
  Atan2 : Trigonometry  Operator=atan2
  Constant : Constant  Value=2*pi  OutDataTypeStr=single
  Constant4 : Constant  Value=sqrt(3)  OutDataTypeStr=single
  Constant5 : Constant  Value=pi/3  OutDataTypeStr=single
  Demux : Demux  Outputs=3
  Divide : Product  Inputs=*/
  Divide1 : Product  Inputs=*/
  Gain : Gain  Gain=1/2  OutDataTypeStr=single
  Mod : Math  Operator=mod
  Multiport Switch : MultiPortSwitch  Inputs=6  SaturateOnIntegerOverflow=off  InputSameDT=off
  Multiport Switch1 : MultiPortSwitch  Inputs=6  SaturateOnIntegerOverflow=off  InputSameDT=off
  Multiport Switch2 : MultiPortSwitch  Inputs=6  SaturateOnIntegerOverflow=off  InputSameDT=off
  Mux : Mux  Inputs=3
  Normalise Angle : Subsystem
  Product : Product
  Product1 : Product  Inputs=3
  Product2 : Product
  Square : Math  Operator=square
  Square Root : Sqrt
  Square1 : Math  Operator=square
  Trigonometric Function : Trigonometry
  Trigonometric Function1 : Trigonometry
  Da : Outport
  Db : Outport  Port=2
  Dc : Outport  Port=3
  wires:
  Add/1 -> Square Root/1
  Square/1 -> Add/1
  Square1/1 -> Add/2
  Atan2/1 -> Mod/1  "Theta"
  Constant/1 -> Mod/2
  Mod/1 -> Normalise Angle/1(ThetaV)  "ThetaV"
  [V_alpha_ref] -> Atan2/2, Square/1
  [V_beta_ref] -> Atan2/1, Square1/1
  Ts/1 -> [Ts]
  Product1/1 -> Divide/1
  [V_Bus] -> Divide/2
  [Ts] -> Product1/1
  Square Root/1 -> Product1/2  "Vref"
  Constant4/1 -> Product1/3
  Add1/1 -> Trigonometric Function/1
  Normalise Angle/1(Gamma) -> Trigonometric Function1/1, Add1/2
  Constant5/1 -> Add1/1
  Divide/1 -> Product/1, Product2/1
  Trigonometric Function/1 -> Product/2
  Product/1 -> Add3/1, Add2/2, Add5/1  "T1"
  Product2/1 -> Add4/2, Add2/3, Add5/2  "T2"
  Trigonometric Function1/1 -> Product2/2
  [Ts] -> Add2/1
  Add2/1 -> Gain/1  "T0"
  Gain/1 -> Add4/1, Add3/2, [Tz]
  Add3/1 -> [Tx]
  Add4/1 -> [Ty]
  Normalise Angle/2(Sector) -> Multiport Switch2/1, Multiport Switch1/1, Multiport Switch/1
  [Tz] -> Add5/3
  Add5/1 -> [Tw]
  [Tw] -> Multiport Switch/2
  [Tx] -> Multiport Switch/3
  [Tz] -> Multiport Switch/4
  [Tz] -> Multiport Switch/5
  [Ty] -> Multiport Switch/6
  [Tw] -> Multiport Switch/7
  [Ty] -> Multiport Switch1/2
  [Tw] -> Multiport Switch1/4
  [Tw] -> Multiport Switch1/3
  [Tx] -> Multiport Switch1/5
  [Tz] -> Multiport Switch1/6
  [Tz] -> Multiport Switch1/7
  [Tz] -> Multiport Switch2/2
  [Tz] -> Multiport Switch2/3
  [Ty] -> Multiport Switch2/4
  [Tw] -> Multiport Switch2/5
  [Tw] -> Multiport Switch2/6
  [Tx] -> Multiport Switch2/7
  Multiport Switch/1 -> Mux/1  "Ta"
  Multiport Switch1/1 -> Mux/2  "Tb"
  Multiport Switch2/1 -> Mux/3  "Tc"
  Mux/1 -> Divide1/1
  [Ts] -> Divide1/2
  Divide1/1 -> %/1
  Demux/1 -> Da/1
  Demux/2 -> Db/1
  Demux/3 -> Dc/1
  Vα_Ref/1 -> [V_alpha_ref]
  Vβ_Ref/1 -> [V_beta_ref]
  VBus/1 -> [V_Bus]
  %/1 -> Demux/1

== system FOC/50us/Function-Call Subsystem/Phase Current/Enabled Subsystem ==
  " " : Inport
  "  " : Inport  Port=2
  "   " : Inport  Port=3
  Enable : EnablePort
  IPhaseU : Outport
  IPhaseV : Outport  Port=2
  IPhaseW : Outport  Port=3
  wires:
  " "/1 -> IPhaseU/1
  "  "/1 -> IPhaseV/1
  "   "/1 -> IPhaseW/1

== system FOC/50us/Function-Call Subsystem/FOC/Sector Based SVPWM/Normalise Angle ==
  note: Gamma - Angle within the sector
      | Must be between 0 - 60 degrees
  note: Sector: how many ThetaV can
      | pi/3 (60 degrees) contain
  ThetaV : Inport
  Add : Sum  Inputs=+-
  Add Constant : Bias  Bias=1  SaturateOnIntegerOverflow=off
  Constant : Constant  Value=pi/3  OutDataTypeStr=single
  Constant1 : Constant  Value=pi/3  OutDataTypeStr=single
  Data Type Conversion : DataTypeConversion  OutDataTypeStr=uint8  SaturateOnIntegerOverflow=off  RndMeth=Floor
  Divide : Product  Inputs=*/
  Floor : Rounding
  Product : Product
  Gamma : Outport
  Sector : Outport  Port=2
  wires:
  ThetaV/1 -> Add/1, Divide/1
  Constant/1 -> Divide/2
  Divide/1 -> Floor/1
  Floor/1 -> Add Constant/1, Product/2
  Add Constant/1 -> Data Type Conversion/1
  Add/1 -> Gamma/1
  Constant1/1 -> Product/1
  Product/1 -> Add/2
  Data Type Conversion/1 -> Sector/1
